simulink model "model1_pred_dodatno_20261104_144119"  (R2026a)
settings: Solver=VariableStepAuto  StopTime=60
undefined symbols (not defined in the file or in its folder): m, n
libraries: simulink x3
settings Model: Creator=nejcr  LastModifiedBy=nejcr

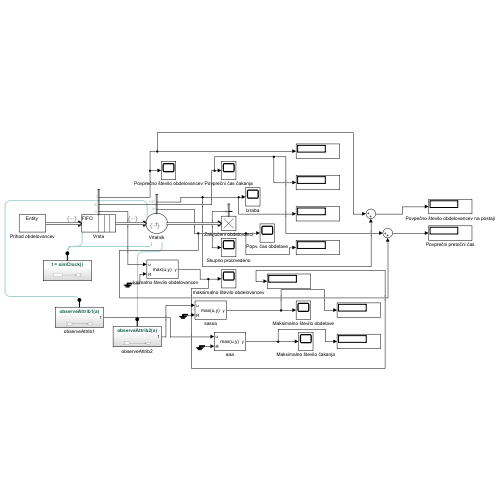
[thumbnail: Simulink's stored preview of the top-level diagram]
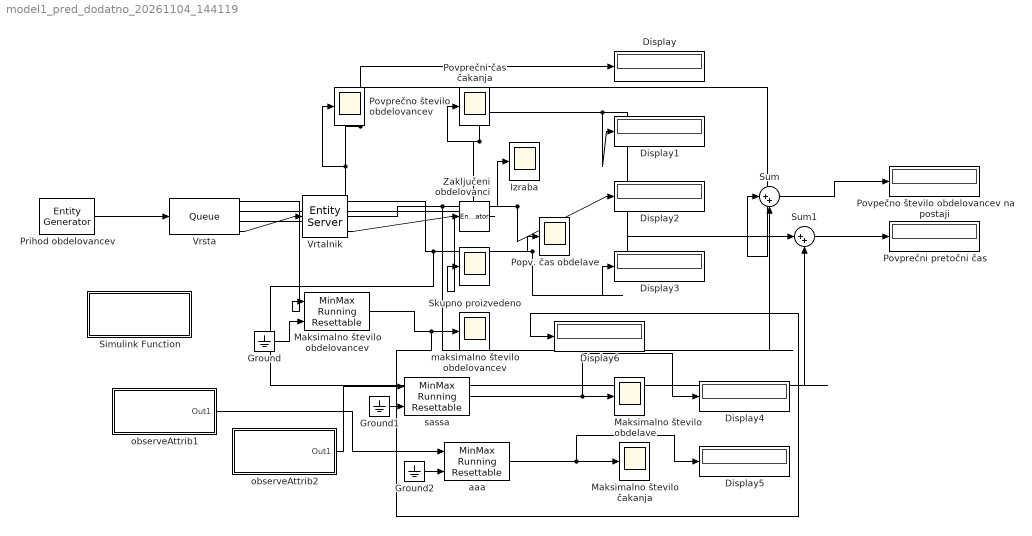
== system model1_pred_dodatno_20261104_144119 ==
  Display{,1..6} (7 alike) : Display
  Ground : Ground
  Ground1 : Ground
  Ground2 : Ground
  Izraba : Scope
      settings: DataLoggingVariableName=ScopeData2
  Maksimalno število obdelave : Scope
      settings: ActiveDisplayYMinimum=-1  ActiveDisplayYMaximum=1  DataLoggingVariableName=ScopeData4
  Maksimalno število obdelovancev : simulink/Math Operations/MinMax Running Resettable  Function=max  vinit=0.0
  Maksimalno število čakanja : Scope
      settings: ActiveDisplayYMinimum=-1  ActiveDisplayYMaximum=1  DataLoggingVariableName=ScopeData6
  Popv. čas obdelave : Scope
      settings: ActiveDisplayYMinimum=-1  ActiveDisplayYMaximum=1  DataLoggingVariableName=ScopeData3
  Povpečno število obdelovancev na postaji : Display
  Povprečni pretočni čas : Display
  Povprečni čas čakanja : Scope
      settings: ActiveDisplayYMinimum=1.7865081354119217  ActiveDisplayYMaximum=4.5093764342368647
  Povprečno število obdelovancev : Scope
      settings: ActiveDisplayYMinimum=-1  ActiveDisplayYMaximum=1
  Prihod obdelovancev : EntityGenerator  OutputPortMessageModes=m  TimeSource=MATLAB action  IntergenerationTimeAction=|  AttributeName=casVstopa|casCakanja|casObdelave  AttributeInitialValue=0|0|0  EntityType=Structured  EntityTypeName=Entity
      | persistent rngInit;
      | if isempty(rngInit)
      |     seed = 12345;
      |     rng(seed);
      |     rngInit = true;
      | end
      | 
      | % Pattern: Expontential distribution
      | mu = 3;
      | dt = -mu * log(1-rand());
  Simulink Function : Subsystem  TreatAsAtomicUnit=on
  Skupno proizvedeno : Scope
      settings: DataLoggingVariableName=ScopeData5
  Sum : Sum  Inputs=|++
  Sum1 : Sum  Inputs=|++
  Vrsta : Queue  InputPortMessageModes=m  OutputPortMessageModes=n,n,n,m  EntryAction=entity.casVstopa=simClock;  NumberEntitiesInBlock=on  AverageWait=on  AverageQueueLength=on
      settings: OutputPortMap=o1,o2,o3,o5
  Vrtalnik : EntityServer  InputPortMessageModes=m  OutputPortMessageModes=n,n,m  Capacity=1  ServiceTimeSource=MATLAB action  ServiceTimeAction=|  EntryAction=|  ServiceCompleteAction=|  AverageWait=on  Utilization=on
      ServiceTimeAction=|
      | persistent rngInit;
      | if isempty(rngInit)
      | seed = 22345;
      | rng(seed);
      | rngInit = true;
      | 
      | end
      | 
      | %%dt= -(13/6)*log(1-rand());
      | 
      | % generation of triangularly distributed random variates
      | % from uniform distribution
      | % minimum
      | % modus
      | % maximum
      | a =1;
      | c = 1.5;
      | b = 4;
      | u = rand();
      | peak = (c-a)/(b-a);
      | if u <= peak,
      |     x = a+sqrt(u*(b-a)*(c-a));
      | else
      |     x= b-sqrt((1-u)*(b-a)*(b-c));
      | 
      | end;
      | dt = x;
      EntryAction=|
      | entity.casCakanja=simClock()-entity.casVstopa;
      | observeAttrib1(entity.casCakanja);
      ServiceCompleteAction=|
      | entity.casObdelave=simClock()-entity.casVstopa-entity.casCakanja;
      | observeAttrib2(entity.casObdelave);
      settings: OutputPortMap=o4,o5,o9
  Zaključeni obdelovanci : EntityTerminator  InputPortMessageModes=m  NumberEntitiesArrived=on
      settings: OutputPortMap=o0
  aaa : simulink/Math Operations/MinMax Running Resettable  Function=max  vinit=0.0
  maksimalno število obdelovancev : Scope
      settings: ActiveDisplayYMinimum=-1  ActiveDisplayYMaximum=1  DataLoggingVariableName=ScopeData7
  observeAttrib1 : Subsystem  TreatAsAtomicUnit=on
  observeAttrib2 : Subsystem  TreatAsAtomicUnit=on
  sassa : simulink/Math Operations/MinMax Running Resettable  Function=max  vinit=0.0
  wires:
  Prihod obdelovancev/1 -> Vrsta/1
  Vrsta/4 -> Vrtalnik/1
  Vrtalnik/3 -> Zaključeni obdelovanci/1
  Ground/1 -> Maksimalno število obdelovancev/2
  Vrsta/3 -> Sum/1, Display/1, Povprečno število obdelovancev/1
  Vrsta/2 -> Sum1/1, Display1/1, Povprečni čas čakanja/1
  Vrsta/1 -> Maksimalno število obdelovancev/1
  Vrtalnik/2 -> Sum/2, Display2/1, Izraba/1
  Vrtalnik/1 -> Sum1/2, Display3/1, Popv. čas obdelave/1
  Zaključeni obdelovanci/1 -> Skupno proizvedeno/1
  Maksimalno število obdelovancev/1 -> Display6/1, maksimalno število obdelovancev/1
  sassa/1 -> Display4/1, Maksimalno število obdelave/1
  aaa/1 -> Display5/1, Maksimalno število čakanja/1
  Ground2/1 -> aaa/2
  Ground1/1 -> sassa/2
  Sum1/1 -> Povprečni pretočni čas/1
  Sum/1 -> Povpečno število obdelovancev na postaji/1
  observeAttrib1/1(Out1) -> aaa/1
  observeAttrib2/1(Out1) -> sassa/1

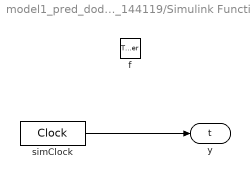
== system model1_pred_dodatno_20261104_144119/Simulink Function ==
  f : TriggerPort  TriggerType=function-call  IsSimulinkFunction=on  FunctionName=simClock  FunctionVisibility=scoped  VariantControl=(inherit)
  simClock : DigitalClock  SampleTime=-1
  y : ArgOut  DisableCoverage=on  ArgumentName=t
  wires:
  simClock/1 -> y/1

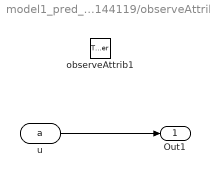
== system model1_pred_dodatno_20261104_144119/observeAttrib1 ==
  observeAttrib1 : TriggerPort  TriggerType=function-call  IsSimulinkFunction=on  FunctionName=observeAttrib1  FunctionVisibility=scoped  VariantControl=(inherit)
  u : ArgIn  DisableCoverage=on  ArgumentName=a
  Out1 : Outport
  wires:
  u/1 -> Out1/1

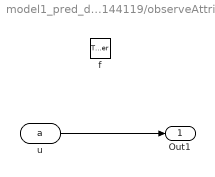
== system model1_pred_dodatno_20261104_144119/observeAttrib2 ==
  f : TriggerPort  TriggerType=function-call  IsSimulinkFunction=on  FunctionName=observeAttrib2  FunctionVisibility=scoped  VariantControl=(inherit)
  u : ArgIn  DisableCoverage=on  ArgumentName=a
  Out1 : Outport
  wires:
  u/1 -> Out1/1
